simulink model "LabPsu_plant"  (R2026b)
values from neighbouring files (symbols this model uses):
  C = double(C)    [labpsu_discrete_plant_coeffs.m]    (also in plant.sldd = 0.0001)
  L = double(L)    [labpsu_discrete_plant_coeffs.m]    (also in plant.sldd = 1.0E-5)
  R = double(R)    [labpsu_discrete_plant_coeffs.m]    (also in plant.sldd = 5.0)
  RL = double(RL)    [labpsu_discrete_plant_coeffs.m]    (also in plant.sldd = 0.001)
  Vin = double(Vin)    [labpsu_discrete_plant_coeffs.m]    (also in plant.sldd = 24.0)
settings Model: Creator=BenjaminRupp  LastModifiedBy=BenjaminRupp

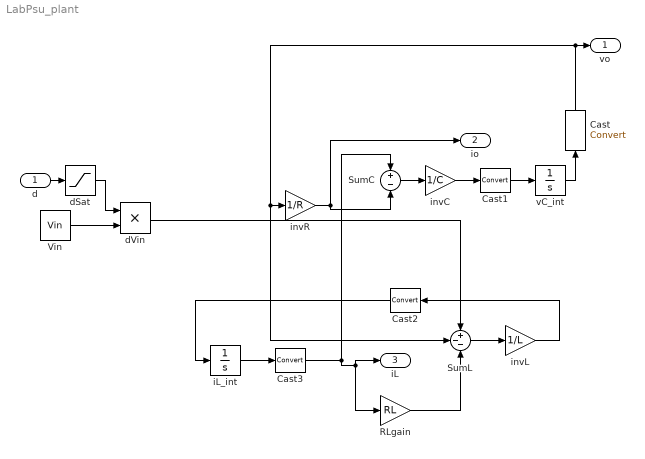
== system LabPsu_plant ==
  d : Inport  OutDataTypeStr=single
  Cast{,1..3} (4 alike) : DataTypeConversion  SaturateOnIntegerOverflow=off  RndMeth=Floor
  RLgain : Gain  Gain=RL  OutDataTypeStr=single
  SumC : Sum  Inputs=+-
  SumL : Sum  Inputs=+--
  Vin : Constant  Value=Vin  OutDataTypeStr=single
  dSat : Saturate  UpperLimit=1  LowerLimit=0
  dVin : Product
  iL_int : Integrator  LimitOutput=on  LowerSaturationLimit=0
  invC : Gain  Gain=1/C  OutDataTypeStr=single
  invL : Gain  Gain=1/L
  invR : Gain  Gain=1/R  OutDataTypeStr=single
  vC_int : Integrator
  vo : Outport  OutDataTypeStr=single
  io : Outport  Port=2  OutDataTypeStr=single
  iL : Outport  Port=3  OutDataTypeStr=single
  wires:
  dSat/1 -> dVin/1
  vC_int/1 -> Cast/1
  d/1 -> dSat/1
  invL/1 -> Cast2/1
  iL_int/1 -> Cast3/1
  invR/1 -> io/1, SumC/2
  Vin/1 -> dVin/2
  dVin/1 -> SumL/1
  RLgain/1 -> SumL/3
  SumL/1 -> invL/1
  Cast/1 -> SumL/2, invR/1, vo/1
  Cast2/1 -> iL_int/1
  Cast3/1 -> iL/1, RLgain/1, SumC/1
  SumC/1 -> invC/1
  invC/1 -> Cast1/1
  Cast1/1 -> vC_int/1
